simulink model "Controller_BMS"  (R2024a)
settings: Solver=FixedStepDiscrete  StartTime=0.0  StopTime=1800  FixedStep=0.01  RelTol=1e-3  EnableMultiTasking=on
InitFcn:
  | init_bms;
values from neighbouring files (symbols this model uses):
  SOC_init = single(0.95)    [init_bms.m]
settings Model: Creator=Lenovo  LastModifiedBy=Lenovo
settings DataIOCC: ExternalInput=ds_in  LoadExternalInput=on  SaveOutput=off  SaveTime=off
settings OptimizationCC: EnhancedBackFolding=on  PassReuseOutputArgsAs=Individual arguments  ZeroExternalMemoryAtStartup=off  ZeroInternalMemoryAtStartup=off  MaxStackSize=64  OptimizeBlockOrder=speed  DifferentSizesBufferReuse=on  OptimizationCustomize=off  EfficientTunableParamExpr=on
settings DebuggingCC: ParameterTunabilityLossMsg=error
settings HardwareCC: ProdBitPerPointer=32  ProdBitPerSizeT=32  ProdBitPerPtrDiffT=32  ProdLargestAtomicInteger=Long  ProdLargestAtomicFloat=Double  ProdWordSize=32  ProdLongLongMode=on  ProdHWDeviceType=ARM Compatible->ARM Cortex-M
settings SFSimCC: MATLABDynamicMemAlloc=off
settings RTWCC: Description=Embedded Coder  SystemTargetFile=ert.tlc  HardwareBoard=STM32L4xx Based  GenCodeOnly=on  TemplateMakefile=ert_default_tmf  Toolchain=GNU Tools for ARM Embedded Processors  CodeExecutionProfiling=on
settings CodeAppCC: ForceParamTrailComments=on  IgnoreCustomStorageClasses=off  OperatorAnnotations=on  SimulinkDataObjDesc=on  SFDataObjDesc=on  InsertBlockDesc=on
settings ERTTargetCC: TargetLangStandard=C99 (ISO)  CodeReplacementLibrary=ARM Cortex-M  ExtModeTransport=3  ExtModeStaticAlloc=on  ExtModeStaticAllocSize=2048  ExtModeMexFile=ext_xcp  ExtModeIntrfLevel=Level2 - Open
settings ConfigComp: CovEnable=on  CovScope=ReferencedModels  RecordCoverage=on  CovMetricSettings=dcm

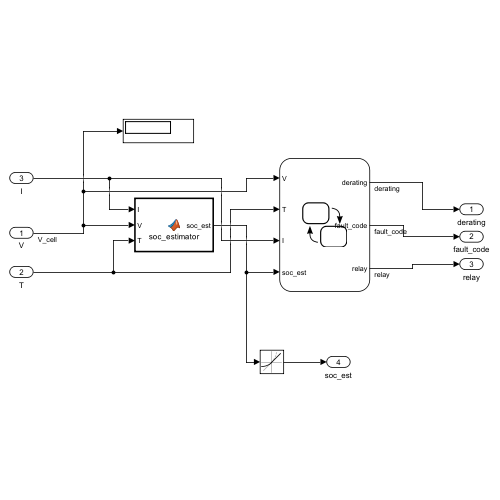
[thumbnail: Simulink's stored preview of the top-level diagram]
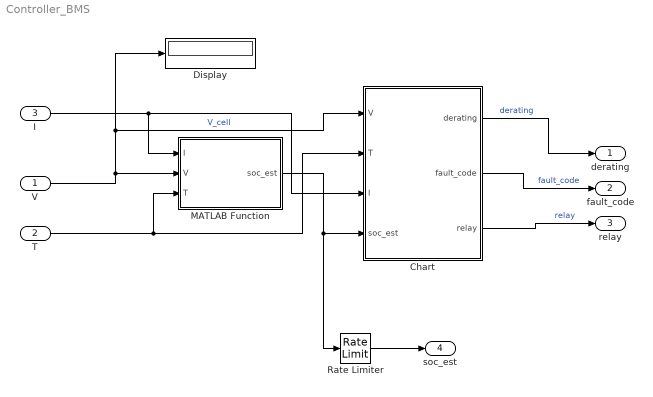
== system Controller_BMS ==
  V : Inport  OutDataTypeStr=single  PortDimensions=1  SampleTime=0.01
  T : Inport  Port=2  OutDataTypeStr=single  PortDimensions=1  SampleTime=0.01
  I : Inport  Port=3  OutDataTypeStr=single  PortDimensions=1  SampleTime=0.01
  Chart : Stateflow chart  TreatAsAtomicUnit=on
  Display : Display
  MATLAB Function : MATLAB Function  TreatAsAtomicUnit=on
  Rate Limiter : RateLimiter  RisingSlewLimit=1e-3  FallingSlewLimit=-1e-3  SampleTimeMode=inherited  InitialCondition=SOC_init
  derating : Outport  OutDataTypeStr=boolean  PortDimensions=1  SampleTime=0.01
  fault_code : Outport  Port=2  OutDataTypeStr=boolean  PortDimensions=1  SampleTime=0.01
  relay : Outport  Port=3  OutDataTypeStr=boolean  PortDimensions=1  SampleTime=0.01
  soc_est : Outport  Port=4  OutDataTypeStr=single  PortDimensions=1  SampleTime=0.01
  wires:
  T/1 -> Chart/2(T), MATLAB Function/3(T)
  Chart/1(derating) -> derating/1  "derating"
  MATLAB Function/1(soc_est) -> Chart/4(soc_est), Rate Limiter/1
  V/1 -> Chart/1(V), Display/1, MATLAB Function/2(V)  "V_cell"
  I/1 -> Chart/3(I), MATLAB Function/1(I)
  Chart/2(fault_code) -> fault_code/1  "fault_code"
  Chart/3(relay) -> relay/1  "relay"
  Rate Limiter/1 -> soc_est/1

== matlab function Controller_BMS/MATLAB Function ==
  data: I input; soc_est output; V input; T input
function soc_est = soc_estimator(I, V, T)
%#codegen
persistent prev
RATE = single(1e-3);   % 1/s, max SOC change rate
TS   = single(0.01);   % sample time

u = double([I; V; T]);
soc_raw = soc_nn_core(u);
soc_nn  = single(min(max(soc_raw, 0.0), 1.0));

if isempty(prev)
    prev = soc_nn;     % init from first estimate
end
step = min(max(soc_nn - prev, -RATE*TS), RATE*TS);
prev = prev + step;
soc_est = prev;
end

== stateflow chart Controller_BMS/Chart ==
  settings: updateMethod=DISCRETE  sampleTime=0.01
  state INIT
    entry :
    relay=0;
    derating=0;
    fault_code=0;
  state NORMAL
    entry:
    relay=1;
    derating=0;
    fault_code=0;
  state DERATING
    entry:
    relay=1;
    derating=1;
    fault_code=0;
  state EMERGENCY_STOP
    entry:
    relay=0;
    derating=0;
    fault_code=1;
  (default) -> INIT
  INIT -> NORMAL : [after(10, tick)]
  NORMAL -> EMERGENCY_STOP [order 1] : [V > 4.25 || V <  2.5 || T >= 55 || I >= 10 ]
  DERATING -> NORMAL [order 2] : [T < 42 && soc_est > 0.20]
  NORMAL -> DERATING [order 2] : [T >= 45 || soc_est <= 0.15 ]
  DERATING -> EMERGENCY_STOP [order 1] : [V > 4.25 || V <  2.5 || T >= 55 || I >= 10]
  data: V input single; T input single; I input single; soc_est input single; derating output boolean; fault_code output boolean; relay output boolean
